simulink model "afe_inv_psm_param"  (R2026b)
settings: Solver=ode23t  StopTime=param.sim.simlength  FixedStep=tc  MaxStep=param.glb_time.tc  RelTol=1e-4
values from neighbouring files (symbols this model uses):
  param = add_template_extras(param, options)    [init_model.m]
undefined symbols (not defined in the file or in its folder): magnitude, omega_m_bez
libraries: fl_lib x330, nesl_utility x174, igbt_simple_2th_lib x12, moving_average_filter x10, moving_average_filter_cc x8, sl_discontinuities x3, single_phase_transformer_lib x3, linear_double_integrator_observer_ccaller x2, discrete_time_low_pass_filter x2, threephase_inductor_lib x2, three_phase_pwm_modulator x2, three_phase_inverter_ideal_switch_based_model x2
(part 8 of 13)

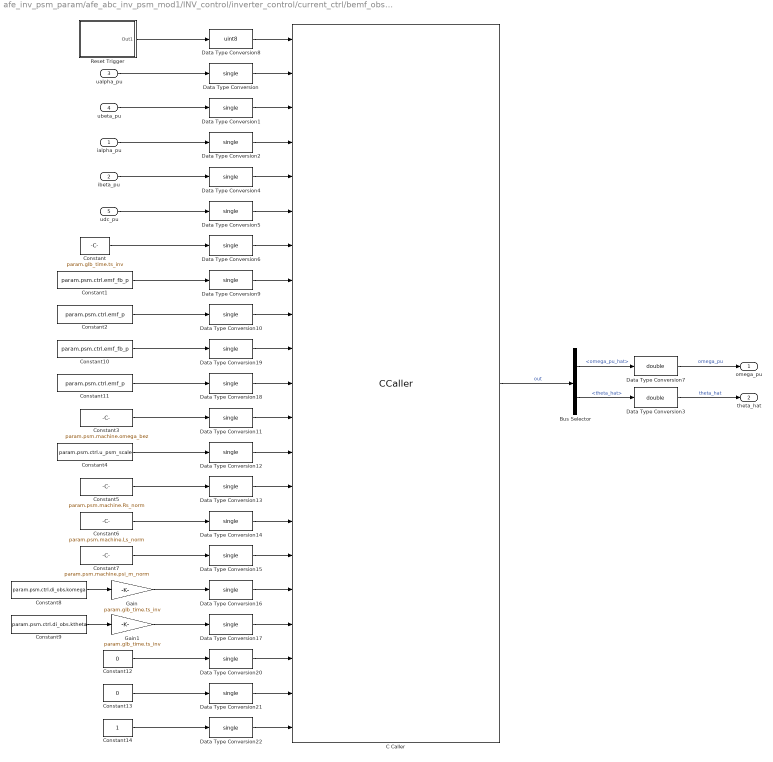
== system afe_inv_psm_param/afe_abc_inv_psm_mod1/INV_control/inverter_control/current_ctrl/bemf_observer/bemf_observer_ccaller ==
  ialpha_pu : Inport
  ibeta_pu : Inport  Port=2
  ualpha_pu : Inport  Port=3
  ubeta_pu : Inport  Port=4
  udc_pu : Inport  Port=5
  Bus Selector : BusSelector  OutputSignals=omega_pu_hat,theta_hat
  C Caller : CCaller  FunctionName=bemf_obsv_process_simulink  PortSpecificationStruct="%)30     .    N\"8   8    (     @         %    \"    !8    !     0         %  0 \"0    $    _    07)G3F%M90  4&]R=$YA;64 4V-O<&4     26YD97@     5'EP90      4VEZ90      27-';&]B86P   X    P    !@    @    $          4    (     0    ,    !         !   P!O=70 #@   #     &    \"     0         !0    @    !     P    $         $  # &]U=  .    .     8    (    !          %    \"     $    &     0         0  ...(+12985 chars)"
  Constant : Constant  Value=param.glb_time.ts_inv
  Constant1 : Constant  Value=param.psm.ctrl.emf_fb_p
  Constant10 : Constant  Value=param.psm.ctrl.emf_fb_p
  Constant11 : Constant  Value=param.psm.ctrl.emf_p
  Constant12 : Constant  Value=0
  Constant13 : Constant  Value=0
  Constant14 : Constant
  Constant2 : Constant  Value=param.psm.ctrl.emf_p
  Constant3 : Constant  Value=param.psm.machine.omega_bez
  Constant4 : Constant  Value=param.psm.ctrl.u_psm_scale
  Constant5 : Constant  Value=param.psm.machine.Rs_norm
  Constant6 : Constant  Value=param.psm.machine.Ls_norm
  Constant7 : Constant  Value=param.psm.machine.psi_m_norm
  Constant8 : Constant  Value=param.psm.ctrl.di_obs.komega
  Constant9 : Constant  Value=param.psm.ctrl.di_obs.ktheta
  Data Type Conversion{,1..2,4..6,9..22} (20 alike) : DataTypeConversion  OutDataTypeStr=single  SaturateOnIntegerOverflow=off  RndMeth=Floor
  Data Type Conversion3 : DataTypeConversion  OutDataTypeStr=double  SaturateOnIntegerOverflow=off  RndMeth=Floor
  Data Type Conversion7 : DataTypeConversion  OutDataTypeStr=double  SaturateOnIntegerOverflow=off  RndMeth=Floor
  Data Type Conversion8 : DataTypeConversion  OutDataTypeStr=uint8  SaturateOnIntegerOverflow=off  RndMeth=Floor
  Gain : Gain  Gain=param.glb_time.ts_inv
  Gain1 : Gain  Gain=param.glb_time.ts_inv
  Reset Trigger : Subsystem
  omega_pu : Outport
  theta_hat : Outport  Port=2
  wires:
  Data Type Conversion5/1 -> C Caller/6
  Data Type Conversion/1 -> C Caller/2
  C Caller/1 -> Bus Selector/1  "out"
  Data Type Conversion1/1 -> C Caller/3
  Data Type Conversion4/1 -> C Caller/5
  Data Type Conversion2/1 -> C Caller/4
  Data Type Conversion6/1 -> C Caller/7
  Bus Selector/2 -> Data Type Conversion3/1  "<theta_hat>"
  Bus Selector/1 -> Data Type Conversion7/1  "<omega_pu_hat>"
  Data Type Conversion7/1 -> omega_pu/1  "omega_pu"
  Data Type Conversion3/1 -> theta_hat/1  "theta_hat"
  Data Type Conversion8/1 -> C Caller/1
  Data Type Conversion9/1 -> C Caller/8
  Data Type Conversion10/1 -> C Caller/9
  Data Type Conversion19/1 -> C Caller/10
  Data Type Conversion18/1 -> C Caller/11
  Data Type Conversion11/1 -> C Caller/12
  Data Type Conversion12/1 -> C Caller/13
  Data Type Conversion13/1 -> C Caller/14
  Data Type Conversion14/1 -> C Caller/15
  Data Type Conversion15/1 -> C Caller/16
  Data Type Conversion16/1 -> C Caller/17
  Data Type Conversion17/1 -> C Caller/18
  Data Type Conversion20/1 -> C Caller/19
  Data Type Conversion21/1 -> C Caller/20
  Data Type Conversion22/1 -> C Caller/21
  Constant14/1 -> Data Type Conversion22/1
  Constant13/1 -> Data Type Conversion21/1
  Constant12/1 -> Data Type Conversion20/1
  Constant9/1 -> Gain1/1
  Constant8/1 -> Gain/1
  Constant7/1 -> Data Type Conversion15/1
  Constant6/1 -> Data Type Conversion14/1
  Constant5/1 -> Data Type Conversion13/1
  Constant4/1 -> Data Type Conversion12/1
  Constant3/1 -> Data Type Conversion11/1
  Constant11/1 -> Data Type Conversion18/1
  Constant10/1 -> Data Type Conversion19/1
  Constant2/1 -> Data Type Conversion10/1
  Constant1/1 -> Data Type Conversion9/1
  Constant/1 -> Data Type Conversion6/1
  ibeta_pu/1 -> Data Type Conversion4/1
  ialpha_pu/1 -> Data Type Conversion2/1
  ubeta_pu/1 -> Data Type Conversion1/1
  ualpha_pu/1 -> Data Type Conversion/1
  Reset Trigger/1(Out1) -> Data Type Conversion8/1
  udc_pu/1 -> Data Type Conversion5/1
  Gain/1 -> Data Type Conversion16/1
  Gain1/1 -> Data Type Conversion17/1

== system afe_inv_psm_param/afe_abc_inv_psm_mod1/INV_control/inverter_control/current_ctrl/current_ctrl/MTPA _mod1 ==
  iq_ref : Inport
  Gain1 : Gain  Gain=1/(param.psm.machine.Ld_norm - param.psm.machine.Lq_norm)/2
  Gain2 : Gain  Gain=1/(param.psm.machine.Ld_norm - param.psm.machine.Lq_norm)/2
  Gain3 : Gain  Gain=-1
  Math Function1 : Math  Operator=magnitude^2  SignedPower=on
  Math Function4 : Math  Operator=magnitude^2  SignedPower=on
  Sqrt : Sqrt
  Sum : Sum  Inputs=|++
  Sum1 : Sum  Inputs=|-+
  id_ref_pu < x < 0 : Saturate  UpperLimit=0  LowerLimit=-param.psm.ctrl.id_lim
  Id_ref_mtpa : Outport  VectorParamsAs1DForOutWhenUnconnected=off
  wires:
  Sum1/1 -> Gain3/1
  id_ref_pu < x < 0/1 -> Id_ref_mtpa/1
  Math Function4/1 -> Sum/1
  Math Function1/1 -> Sum/2
  Gain1/1 -> Math Function4/1
  Sum/1 -> Sqrt/1
  Sqrt/1 -> Sum1/2
  iq_ref/1 -> Math Function1/1
  Gain2/1 -> Sum1/1
  [motor_speed_pu_ctrl_mod1] -> Gain1/1, Gain2/1
  Gain3/1 -> id_ref_pu < x < 0/1

== system afe_inv_psm_param/afe_abc_inv_psm_mod1/INV_control/inverter_control/current_ctrl/current_ctrl/dq_pi_with_vector_antiwindup mod1 ==
  id_ref : Inport
  id : Inport  Port=2
  iq_ref : Inport  Port=3
  iq : Inport  Port=4
  udc_pu : Inport  Port=5
  Variant Source : VariantSource  VariantControls={param.psm.impl.use_current_controller_from_simulink_module_1 == 1, param.psm.impl.use_current_controller_from_ccaller_module_1 == 1}
  Variant Source1 : VariantSource  VariantControls={param.psm.impl.use_current_controller_from_simulink_module_1 == 1, param.psm.impl.use_current_controller_from_ccaller_module_1 == 1}
  dq_vector_pi : Subsystem
  dq_vector_pi_ccaller : Subsystem
  simulink/Ccaller VectorPI : Scope  NumInputPorts=2
      settings: ActiveDisplayYMinimum=-0.12579688616096973  ActiveDisplayYMaximum=0.43534495122730732
  ctrl_d_u : Outport
  ctrl_q_u : Outport  Port=2
  wires:
  id/1 -> dq_vector_pi_ccaller/1(id), dq_vector_pi/1(id)  "id"
  id_ref/1 -> dq_vector_pi_ccaller/2(id_ref), dq_vector_pi/2(id_ref)  "id_ref"
  iq/1 -> dq_vector_pi_ccaller/3(iq), dq_vector_pi/3(iq)  "iq"
  iq_ref/1 -> dq_vector_pi_ccaller/4(iq_ref), dq_vector_pi/4(iq_ref)  "iq_ref"
  dq_vector_pi/1(md_sat) -> Variant Source/1
  dq_vector_pi_ccaller/2(uq_ctrl_out) -> Variant Source1/2
  dq_vector_pi/2(mq_sat) -> Variant Source1/1
  dq_vector_pi_ccaller/1(ud_ctrl_out) -> Variant Source/2
  Variant Source/1 -> ctrl_d_u/1, simulink/Ccaller VectorPI/1  "ctrl_d_u"
  Variant Source1/1 -> simulink/Ccaller VectorPI/2, ctrl_q_u/1  "ctrl_q_u"
  udc_pu/1 -> dq_vector_pi_ccaller/5(udc_pu)

== system afe_inv_psm_param/afe_abc_inv_psm_mod1/INV_control/inverter_control/current_ctrl/current_ctrl/id_ref _mod1 ==
  id_mtpa : Inport
  Constant : Constant  Value=0
  Variant Source : VariantSource  VariantControls={param.psm.mode.use_mtpa == 1, param.psm.mode.use_mtpa == 0}
  id_ref : Outport
  wires:
  Variant Source/1 -> id_ref/1
  id_mtpa/1 -> Variant Source/1
  Constant/1 -> Variant Source/2

== system afe_inv_psm_param/afe_abc_inv_psm_mod1/INV_control/inverter_control/current_ctrl/current_ctrl/output voltage transformation ==
  Unit Delay2 : UnitDelay  SampleTime=-1
  Unit Delay3 : UnitDelay  SampleTime=-1
  dq2alphabeta : MATLAB Function  TreatAsAtomicUnit=on
  tag scope: ualpha_pu_mod1=scoped, ubeta_pu_mod1=scoped
  wires:
  [ud_pu_mod1] -> dq2alphabeta/1(d)
  [uq_pu_mod1] -> dq2alphabeta/2(q)
  Unit Delay2/1 -> [ualpha_pu_mod1]
  dq2alphabeta/2(beta) -> Unit Delay3/1
  Unit Delay3/1 -> [ubeta_pu_mod1]
  dq2alphabeta/1(alpha) -> Unit Delay2/1
  [motor_phase_ctrl_mod1] -> dq2alphabeta/3(gamma)

== system afe_inv_psm_param/afe_abc_inv_psm_mod1/INV_control/inverter_control/phase_compensation_1/alignment_ctrl/pi ==
  u_ref : Inport
  u : Inport  Port=2
  1/Ti : Gain  Gain=kp  SaturateOnIntegerOverflow=on  OutDataTypeStr=Inherit: Same as input  ParamDataTypeStr=Inherit: Same as input
  Saturation : Saturate  UpperLimit=lim_up  LowerLimit=lim_down
  Sum1 : Sum  Inputs=+++  SaturateOnIntegerOverflow=on
  Sum2 : Sum  Inputs=-+  SaturateOnIntegerOverflow=on
  Sum3 : Sum  Inputs=-+  SaturateOnIntegerOverflow=on
  Unit Delay4 : UnitDelay  SampleTime=-1
  kp : Gain  Gain=ki  SaturateOnIntegerOverflow=on  OutDataTypeStr=Inherit: Same as input  ParamDataTypeStr=Inherit: Same as input
  y : Outport
  wires:
  1/Ti/1 -> Sum1/1, Sum3/1
  kp/1 -> Sum1/2
  Sum3/1 -> Unit Delay4/1
  Unit Delay4/1 -> Sum1/3
  u_ref/1 -> Sum2/2
  u/1 -> Sum2/1
  Sum2/1 -> kp/1, 1/Ti/1
  Sum1/1 -> Saturation/1
  Saturation/1 -> Sum3/2, y/1

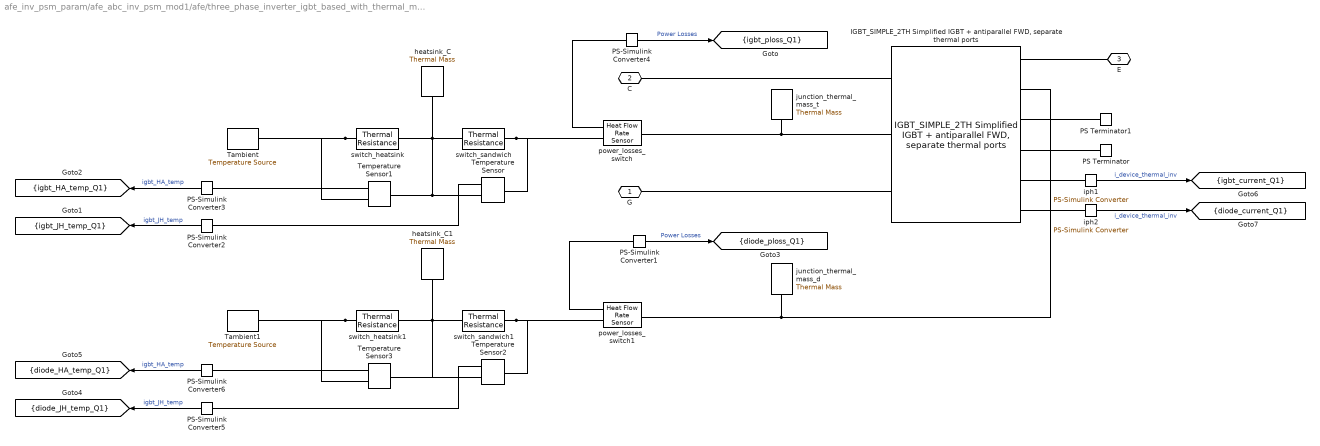
== system afe_inv_psm_param/afe_abc_inv_psm_mod1/afe/three_phase_inverter_igbt_based_with_thermal_model/three_phase_inverter_with_igbt_simple_2th/igbt_simple_1/IGBT_simple ==
  "IGBT_SIMPLE_2TH Simplified IGBT + antiparallel FWD, separate thermal ports" : igbt_simple_2th_lib/IGBT_SIMPLE_2TH Simplified IGBT + antiparallel FWD, separate thermal ports  Vce_sat=vce_sat_m V  Vf=v_gamma_m V  Vth=Vth_gate_m V  Vhyst=Vth_gate_hyst_m V  Eon_ref=Eon_m mJ  Eoff_ref=Eoff_m mJ  Err_ref=Err_m mJ  Ic_ref=Ic_ref_m A  Vdc_ref=Vdc_ref_m V  V_rr_th=Vblock_Errf_m V  Ron=rce_on_m mOhm  Rd=rd_on_m mOhm  Goff=Gce_off_m 1/Ohm  tau_s=time_constant_edge_m us  tau_p=time_constant_ploss_m us  i_specify=off  i_priority=None  i=0 A  i_nominal_specify=off  i_nominal_value=1  i_nominal_unit=A  v_specify=off  v_priority=None  v=0 V  v_nominal_specify=off  v_nominal_value=1  v_nominal_unit=V  i_t_specify=off  i_t_priority=None  i_t=0 A  i_t_nominal_specify=off  i_t_nominal_value=1  i_t_nominal_unit=A  i_d_specify=off  i_d_priority=None  i_d=0 A  i_d_nominal_specify=off  i_d_nominal_value=1  i_d_nominal_unit=A  i_h_specify=off  i_h_priority=None  i_h=0 A  i_h_nominal_specify=off  i_h_nominal_value=1  i_h_nominal_unit=A  i_dh_specify=off  i_dh_priority=None  i_dh=0 A  i_dh_nominal_specify=off  i_dh_nominal_value=1  i_dh_nominal_unit=A  v_h_specify=off  v_h_priority=None  v_h=0 V  v_h_nominal_specify=off  v_h_nominal_value=1  v_h_nominal_unit=V  E_lpt_specify=off  E_lpt_priority=None  E_lpt=0 J  E_lpt_nominal_specify=off  E_lpt_nominal_value=1  E_lpt_nominal_unit=J  E_lpd_specify=off  E_lpd_priority=None  E_lpd=0 J  E_lpd_nominal_specify=off  E_lpd_nominal_value=1  E_lpd_nominal_unit=J  Qt_specify=off  Qt_priority=None  Qt=0 W  Qt_nominal_specify=off  Qt_nominal_value=1  Qt_nominal_unit=W  Qd_specify=off  Qd_priority=None  Qd=0 W  Qd_nominal_specify=off  Qd_nominal_value=1  Qd_nominal_unit=W  E_t_specify=off  E_t_priority=None  E_t=0 J  E_d_specify=off  E_d_priority=None  E_d=0 J
  PS Terminator : fl_lib/Physical Signals/Sinks/PS Terminator
  PS Terminator1 : fl_lib/Physical Signals/Sinks/PS Terminator
  PS-Simulink Converter1 : nesl_utility/PS-Simulink Converter  PhysicalDomain=network_engine_domain  SubClassName=ps_output  LeftPortType=input  RightPortType=output  PseudoPeriodic=off  Frequencies=[]  VectorFormat=1-D array  Unit=J/s  AffineConversion=off
  PS-Simulink Converter{2..3,5..6} (4 alike) : nesl_utility/PS-Simulink Converter  PhysicalDomain=network_engine_domain  SubClassName=ps_output  LeftPortType=input  RightPortType=output  PseudoPeriodic=off  Frequencies=[]  VectorFormat=1-D array  Unit=degC  AffineConversion=off
  PS-Simulink Converter4 : nesl_utility/PS-Simulink Converter  PhysicalDomain=network_engine_domain  SubClassName=ps_output  LeftPortType=input  RightPortType=output  PseudoPeriodic=off  Frequencies=[]  VectorFormat=1-D array  Unit=J/s  AffineConversion=off
  Tambient : fl_lib/Thermal/Thermal Sources/Temperature Source  temperature=Tambient_m degC
  Tambient1 : fl_lib/Thermal/Thermal Sources/Temperature Source  temperature=Tambient_m degC
  Temperature Sensor{,1..3} (4 alike) : fl_lib/Thermal/Thermal Sensors/Temperature Sensor  temperature_measure=foundation.enum.MeasurementReference.difference
  heatsink_C : fl_lib/Thermal/Thermal Elements/Thermal Mass  mass_type=foundation.enum.constant_variable.constant  mass=mass_heatsink_m kg  sp_heat=specific_heat_m J/(K*kg)  mass_min=1e-6 kg  num_ports=foundation.enum.numPorts2.one  m_specify=off  m_priority=High  m=1 kg  m_nominal_specify=off  m_nominal_value=1  m_nominal_unit=kg  T_specify=on  T_priority=High  T=Tambient_m degC  T_nominal_specify=off  T_nominal_value=1  T_nominal_unit=K  Q_specify=off  Q_priority=High  Q=0 W  Q_nominal_specify=off  Q_nominal_value=1  Q_nominal_unit=W
  heatsink_C1 : fl_lib/Thermal/Thermal Elements/Thermal Mass  mass_type=foundation.enum.constant_variable.constant  mass=mass_heatsink_m kg  sp_heat=specific_heat_m J/(K*kg)  mass_min=1e-6 kg  num_ports=foundation.enum.numPorts2.one  m_specify=off  m_priority=High  m=1 kg  m_nominal_specify=off  m_nominal_value=1  m_nominal_unit=kg  T_specify=on  T_priority=High  T=Tambient_m degC  T_nominal_specify=off  T_nominal_value=1  T_nominal_unit=K  Q_specify=off  Q_priority=High  Q=0 W  Q_nominal_specify=off  Q_nominal_value=1  Q_nominal_unit=W
  iph1 : nesl_utility/PS-Simulink Converter  PhysicalDomain=network_engine_domain  SubClassName=ps_output  LeftPortType=input  RightPortType=output  PseudoPeriodic=off  Frequencies=[]  VectorFormat=1-D array  Unit=A  AffineConversion=off
  iph2 : nesl_utility/PS-Simulink Converter  PhysicalDomain=network_engine_domain  SubClassName=ps_output  LeftPortType=input  RightPortType=output  PseudoPeriodic=off  Frequencies=[]  VectorFormat=1-D array  Unit=A  AffineConversion=off
  junction_thermal_mass_d : fl_lib/Thermal/Thermal Elements/Thermal Mass  mass_type=foundation.enum.constant_variable.constant  mass=JunctionTermalMass_m/specific_heat_m kg  sp_heat=specific_heat_m J/(K*kg)  mass_min=1e-6 kg  num_ports=foundation.enum.numPorts2.one  m_specify=off  m_priority=High  m=1 kg  m_nominal_specify=off  m_nominal_value=1  m_nominal_unit=kg  T_specify=on  T_priority=High  T=Tambient_m degC  T_nominal_specify=off  T_nominal_value=1  T_nominal_unit=K  Q_specify=off  Q_priority=High  Q=0 W  Q_nominal_specify=off  Q_nominal_value=1  Q_nominal_unit=W
  junction_thermal_mass_t : fl_lib/Thermal/Thermal Elements/Thermal Mass  mass_type=foundation.enum.constant_variable.constant  mass=JunctionTermalMass_m/specific_heat_m kg  sp_heat=specific_heat_m J/(K*kg)  mass_min=1e-6 kg  num_ports=foundation.enum.numPorts2.one  m_specify=off  m_priority=High  m=1 kg  m_nominal_specify=off  m_nominal_value=1  m_nominal_unit=kg  T_specify=on  T_priority=High  T=Tambient_m degC  T_nominal_specify=off  T_nominal_value=1  T_nominal_unit=K  Q_specify=off  Q_priority=High  Q=0 W  Q_nominal_specify=off  Q_nominal_value=1  Q_nominal_unit=W
  power_losses_switch : fl_lib/Thermal/Thermal Sensors/Heat Flow Rate Sensor
  power_losses_switch1 : fl_lib/Thermal/Thermal Sensors/Heat Flow Rate Sensor
  switch_heatsink : fl_lib/Thermal/Thermal Elements/Thermal Resistance  resistance=rth_switch_HA_m K/W  T_specify=off  T_priority=High  T=0 deltadegC  T_nominal_specify=off  T_nominal_value=1  T_nominal_unit=K  Q_specify=off  Q_priority=None  Q=0 W  Q_nominal_specify=off  Q_nominal_value=1  Q_nominal_unit=W
  switch_heatsink1 : fl_lib/Thermal/Thermal Elements/Thermal Resistance  resistance=rth_diode_HA_m K/W  T_specify=off  T_priority=High  T=0 deltadegC  T_nominal_specify=off  T_nominal_value=1  T_nominal_unit=K  Q_specify=off  Q_priority=None  Q=0 W  Q_nominal_specify=off  Q_nominal_value=1  Q_nominal_unit=W
  switch_sandwich : fl_lib/Thermal/Thermal Elements/Thermal Resistance  resistance=rth_switch_JH_m K/W  T_specify=off  T_priority=High  T=0 degC  T_nominal_specify=off  T_nominal_value=1  T_nominal_unit=K  Q_specify=off  Q_priority=None  Q=0 W  Q_nominal_specify=off  Q_nominal_value=1  Q_nominal_unit=W
  switch_sandwich1 : fl_lib/Thermal/Thermal Elements/Thermal Resistance  resistance=rth_diode_JH_m K/W  T_specify=off  T_priority=High  T=0 degC  T_nominal_specify=off  T_nominal_value=1  T_nominal_unit=K  Q_specify=off  Q_priority=None  Q=0 W  Q_nominal_specify=off  Q_nominal_value=1  Q_nominal_unit=W
  G : PMIOPort  Side=Left
  C : PMIOPort  Port=2  Side=Left
  E : PMIOPort  Port=3  Side=Right
  tag scope: diode_HA_temp_Q1=scoped, diode_JH_temp_Q1=scoped, diode_current_Q1=scoped, diode_ploss_Q1=scoped, igbt_HA_temp_Q1=scoped, igbt_JH_temp_Q1=scoped, igbt_current_Q1=scoped, igbt_ploss_Q1=scoped
  wires:
  PS-Simulink Converter3/1 -> [igbt_HA_temp_Q1]  "igbt_HA_temp"
  PS-Simulink Converter4/1 -> [igbt_ploss_Q1]  "Power Losses"
  PS-Simulink Converter2/1 -> [igbt_JH_temp_Q1]  "igbt_JH_temp"
  PS-Simulink Converter1/1 -> [diode_ploss_Q1]  "Power Losses"
  PS-Simulink Converter5/1 -> [diode_JH_temp_Q1]  "igbt_JH_temp"
  PS-Simulink Converter6/1 -> [diode_HA_temp_Q1]  "igbt_HA_temp"
  iph1/1 -> [igbt_current_Q1]  "i_device_thermal_inv"
  iph2/1 -> [diode_current_Q1]  "i_device_thermal_inv"
  connections:
  Temperature Sensor/RConn2 -- PS-Simulink Converter2/LConn1
  "IGBT_SIMPLE_2TH Simplified IGBT + antiparallel FWD, separate thermal ports"/LConn2 -- junction_thermal_mass_t/LConn1 -- power_losses_switch/LConn1
  Temperature Sensor1/RConn2 -- PS-Simulink Converter3/LConn1
  Temperature Sensor1/LConn1 -- Temperature Sensor/RConn1 -- switch_heatsink/LConn1 -- heatsink_C/LConn1 -- switch_sandwich/RConn1
  switch_heatsink/RConn1 -- Tambient/LConn1 -- Temperature Sensor1/RConn1
  switch_sandwich/LConn1 -- power_losses_switch/RConn2 -- Temperature Sensor/LConn1
  "IGBT_SIMPLE_2TH Simplified IGBT + antiparallel FWD, separate thermal ports"/RConn1 -- E/RConn1
  "IGBT_SIMPLE_2TH Simplified IGBT + antiparallel FWD, separate thermal ports"/LConn1 -- C/RConn1
  "IGBT_SIMPLE_2TH Simplified IGBT + antiparallel FWD, separate thermal ports"/LConn3 -- G/RConn1
  switch_heatsink1/LConn1 -- switch_sandwich1/RConn1 -- heatsink_C1/LConn1 -- Temperature Sensor2/RConn1 -- Temperature Sensor3/LConn1
  switch_heatsink1/RConn1 -- Temperature Sensor3/RConn1 -- Tambient1/LConn1
  switch_sandwich1/LConn1 -- Temperature Sensor2/LConn1 -- power_losses_switch1/RConn2
  Temperature Sensor3/RConn2 -- PS-Simulink Converter6/LConn1
  Temperature Sensor2/RConn2 -- PS-Simulink Converter5/LConn1
  power_losses_switch1/LConn1 -- "IGBT_SIMPLE_2TH Simplified IGBT + antiparallel FWD, separate thermal ports"/RConn2 -- junction_thermal_mass_d/LConn1
  "IGBT_SIMPLE_2TH Simplified IGBT + antiparallel FWD, separate thermal ports"/RConn5 -- iph1/LConn1
  "IGBT_SIMPLE_2TH Simplified IGBT + antiparallel FWD, separate thermal ports"/RConn6 -- iph2/LConn1
  PS Terminator1/LConn1 -- "IGBT_SIMPLE_2TH Simplified IGBT + antiparallel FWD, separate thermal ports"/RConn3
  PS Terminator/LConn1 -- "IGBT_SIMPLE_2TH Simplified IGBT + antiparallel FWD, separate thermal ports"/RConn4
  PS-Simulink Converter4/LConn1 -- power_losses_switch/RConn1
  PS-Simulink Converter1/LConn1 -- power_losses_switch1/RConn1

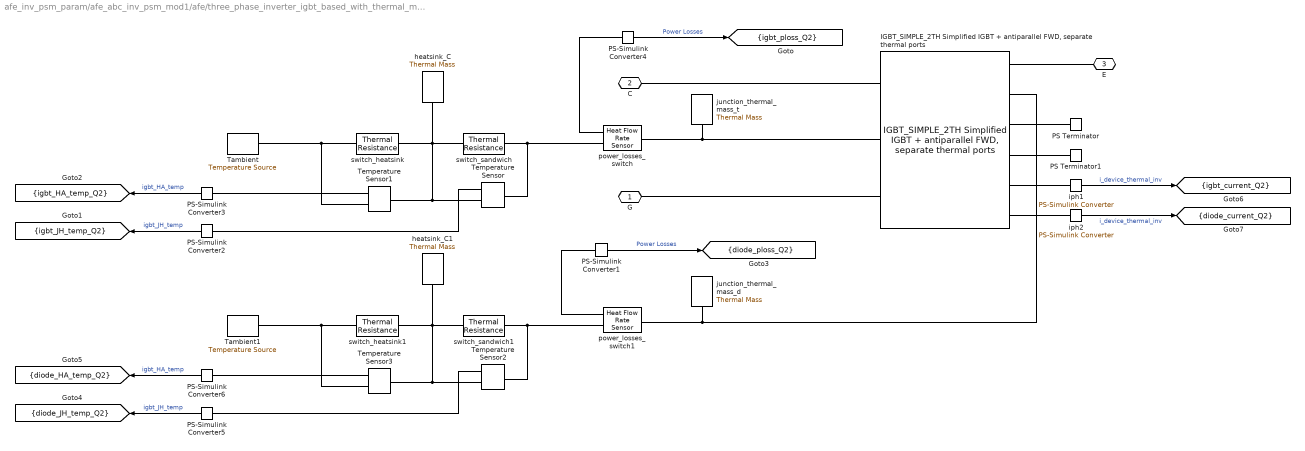
== system afe_inv_psm_param/afe_abc_inv_psm_mod1/afe/three_phase_inverter_igbt_based_with_thermal_model/three_phase_inverter_with_igbt_simple_2th/igbt_simple_2/IGBT_simple ==
  "IGBT_SIMPLE_2TH Simplified IGBT + antiparallel FWD, separate thermal ports" : igbt_simple_2th_lib/IGBT_SIMPLE_2TH Simplified IGBT + antiparallel FWD, separate thermal ports  Vce_sat=vce_sat_m V  Vf=v_gamma_m V  Vth=Vth_gate_m V  Vhyst=Vth_gate_hyst_m V  Eon_ref=Eon_m mJ  Eoff_ref=Eoff_m mJ  Err_ref=Err_m mJ  Ic_ref=Ic_ref_m A  Vdc_ref=Vdc_ref_m V  V_rr_th=Vblock_Errf_m V  Ron=rce_on_m mOhm  Rd=rd_on_m mOhm  Goff=Gce_off_m 1/Ohm  tau_s=time_constant_edge_m us  tau_p=time_constant_ploss_m us  i_specify=off  i_priority=None  i=0 A  i_nominal_specify=off  i_nominal_value=1  i_nominal_unit=A  v_specify=off  v_priority=None  v=0 V  v_nominal_specify=off  v_nominal_value=1  v_nominal_unit=V  i_t_specify=off  i_t_priority=None  i_t=0 A  i_t_nominal_specify=off  i_t_nominal_value=1  i_t_nominal_unit=A  i_d_specify=off  i_d_priority=None  i_d=0 A  i_d_nominal_specify=off  i_d_nominal_value=1  i_d_nominal_unit=A  i_h_specify=off  i_h_priority=None  i_h=0 A  i_h_nominal_specify=off  i_h_nominal_value=1  i_h_nominal_unit=A  i_dh_specify=off  i_dh_priority=None  i_dh=0 A  i_dh_nominal_specify=off  i_dh_nominal_value=1  i_dh_nominal_unit=A  v_h_specify=off  v_h_priority=None  v_h=0 V  v_h_nominal_specify=off  v_h_nominal_value=1  v_h_nominal_unit=V  E_lpt_specify=off  E_lpt_priority=None  E_lpt=0 J  E_lpt_nominal_specify=off  E_lpt_nominal_value=1  E_lpt_nominal_unit=J  E_lpd_specify=off  E_lpd_priority=None  E_lpd=0 J  E_lpd_nominal_specify=off  E_lpd_nominal_value=1  E_lpd_nominal_unit=J  Qt_specify=off  Qt_priority=None  Qt=0 W  Qt_nominal_specify=off  Qt_nominal_value=1  Qt_nominal_unit=W  Qd_specify=off  Qd_priority=None  Qd=0 W  Qd_nominal_specify=off  Qd_nominal_value=1  Qd_nominal_unit=W  E_t_specify=off  E_t_priority=None  E_t=0 J  E_d_specify=off  E_d_priority=None  E_d=0 J
  PS Terminator : fl_lib/Physical Signals/Sinks/PS Terminator
  PS Terminator1 : fl_lib/Physical Signals/Sinks/PS Terminator
  PS-Simulink Converter1 : nesl_utility/PS-Simulink Converter  PhysicalDomain=network_engine_domain  SubClassName=ps_output  LeftPortType=input  RightPortType=output  PseudoPeriodic=off  Frequencies=[]  VectorFormat=1-D array  Unit=J/s  AffineConversion=off
  PS-Simulink Converter{2..3,5..6} (4 alike) : nesl_utility/PS-Simulink Converter  PhysicalDomain=network_engine_domain  SubClassName=ps_output  LeftPortType=input  RightPortType=output  PseudoPeriodic=off  Frequencies=[]  VectorFormat=1-D array  Unit=degC  AffineConversion=off
  PS-Simulink Converter4 : nesl_utility/PS-Simulink Converter  PhysicalDomain=network_engine_domain  SubClassName=ps_output  LeftPortType=input  RightPortType=output  PseudoPeriodic=off  Frequencies=[]  VectorFormat=1-D array  Unit=J/s  AffineConversion=off
  Tambient : fl_lib/Thermal/Thermal Sources/Temperature Source  temperature=Tambient_m degC
  Tambient1 : fl_lib/Thermal/Thermal Sources/Temperature Source  temperature=Tambient_m degC
  Temperature Sensor{,1..3} (4 alike) : fl_lib/Thermal/Thermal Sensors/Temperature Sensor  temperature_measure=foundation.enum.MeasurementReference.difference
  heatsink_C : fl_lib/Thermal/Thermal Elements/Thermal Mass  mass_type=foundation.enum.constant_variable.constant  mass=mass_heatsink_m kg  sp_heat=specific_heat_m J/(K*kg)  mass_min=1e-6 kg  num_ports=foundation.enum.numPorts2.one  m_specify=off  m_priority=High  m=1 kg  m_nominal_specify=off  m_nominal_value=1  m_nominal_unit=kg  T_specify=on  T_priority=High  T=Tambient_m degC  T_nominal_specify=off  T_nominal_value=1  T_nominal_unit=K  Q_specify=off  Q_priority=High  Q=0 W  Q_nominal_specify=off  Q_nominal_value=1  Q_nominal_unit=W
  heatsink_C1 : fl_lib/Thermal/Thermal Elements/Thermal Mass  mass_type=foundation.enum.constant_variable.constant  mass=mass_heatsink_m kg  sp_heat=specific_heat_m J/(K*kg)  mass_min=1e-6 kg  num_ports=foundation.enum.numPorts2.one  m_specify=off  m_priority=High  m=1 kg  m_nominal_specify=off  m_nominal_value=1  m_nominal_unit=kg  T_specify=on  T_priority=High  T=Tambient_m degC  T_nominal_specify=off  T_nominal_value=1  T_nominal_unit=K  Q_specify=off  Q_priority=High  Q=0 W  Q_nominal_specify=off  Q_nominal_value=1  Q_nominal_unit=W
  iph1 : nesl_utility/PS-Simulink Converter  PhysicalDomain=network_engine_domain  SubClassName=ps_output  LeftPortType=input  RightPortType=output  PseudoPeriodic=off  Frequencies=[]  VectorFormat=1-D array  Unit=A  AffineConversion=off
  iph2 : nesl_utility/PS-Simulink Converter  PhysicalDomain=network_engine_domain  SubClassName=ps_output  LeftPortType=input  RightPortType=output  PseudoPeriodic=off  Frequencies=[]  VectorFormat=1-D array  Unit=A  AffineConversion=off
  junction_thermal_mass_d : fl_lib/Thermal/Thermal Elements/Thermal Mass  mass_type=foundation.enum.constant_variable.constant  mass=JunctionTermalMass_m/specific_heat_m kg  sp_heat=specific_heat_m J/(K*kg)  mass_min=1e-6 kg  num_ports=foundation.enum.numPorts2.one  m_specify=off  m_priority=High  m=1 kg  m_nominal_specify=off  m_nominal_value=1  m_nominal_unit=kg  T_specify=on  T_priority=High  T=Tambient_m degC  T_nominal_specify=off  T_nominal_value=1  T_nominal_unit=K  Q_specify=off  Q_priority=High  Q=0 W  Q_nominal_specify=off  Q_nominal_value=1  Q_nominal_unit=W
  junction_thermal_mass_t : fl_lib/Thermal/Thermal Elements/Thermal Mass  mass_type=foundation.enum.constant_variable.constant  mass=JunctionTermalMass_m/specific_heat_m kg  sp_heat=specific_heat_m J/(K*kg)  mass_min=1e-6 kg  num_ports=foundation.enum.numPorts2.one  m_specify=off  m_priority=High  m=1 kg  m_nominal_specify=off  m_nominal_value=1  m_nominal_unit=kg  T_specify=on  T_priority=High  T=Tambient_m degC  T_nominal_specify=off  T_nominal_value=1  T_nominal_unit=K  Q_specify=off  Q_priority=High  Q=0 W  Q_nominal_specify=off  Q_nominal_value=1  Q_nominal_unit=W
  power_losses_switch : fl_lib/Thermal/Thermal Sensors/Heat Flow Rate Sensor
  power_losses_switch1 : fl_lib/Thermal/Thermal Sensors/Heat Flow Rate Sensor
  switch_heatsink : fl_lib/Thermal/Thermal Elements/Thermal Resistance  resistance=rth_switch_HA_m K/W  T_specify=off  T_priority=High  T=0 deltadegC  T_nominal_specify=off  T_nominal_value=1  T_nominal_unit=K  Q_specify=off  Q_priority=None  Q=0 W  Q_nominal_specify=off  Q_nominal_value=1  Q_nominal_unit=W
  switch_heatsink1 : fl_lib/Thermal/Thermal Elements/Thermal Resistance  resistance=rth_diode_HA_m K/W  T_specify=off  T_priority=High  T=0 deltadegC  T_nominal_specify=off  T_nominal_value=1  T_nominal_unit=K  Q_specify=off  Q_priority=None  Q=0 W  Q_nominal_specify=off  Q_nominal_value=1  Q_nominal_unit=W
  switch_sandwich : fl_lib/Thermal/Thermal Elements/Thermal Resistance  resistance=rth_switch_JH_m K/W  T_specify=off  T_priority=High  T=0 degC  T_nominal_specify=off  T_nominal_value=1  T_nominal_unit=K  Q_specify=off  Q_priority=None  Q=0 W  Q_nominal_specify=off  Q_nominal_value=1  Q_nominal_unit=W
  switch_sandwich1 : fl_lib/Thermal/Thermal Elements/Thermal Resistance  resistance=rth_diode_JH_m K/W  T_specify=off  T_priority=High  T=0 degC  T_nominal_specify=off  T_nominal_value=1  T_nominal_unit=K  Q_specify=off  Q_priority=None  Q=0 W  Q_nominal_specify=off  Q_nominal_value=1  Q_nominal_unit=W
  G : PMIOPort  Side=Left
  C : PMIOPort  Port=2  Side=Left
  E : PMIOPort  Port=3  Side=Right
  tag scope: diode_HA_temp_Q2=scoped, diode_JH_temp_Q2=scoped, diode_current_Q2=scoped, diode_ploss_Q2=scoped, igbt_HA_temp_Q2=scoped, igbt_JH_temp_Q2=scoped, igbt_current_Q2=scoped, igbt_ploss_Q2=scoped
  wires:
  iph2/1 -> [diode_current_Q2]  "i_device_thermal_inv"
  iph1/1 -> [igbt_current_Q2]  "i_device_thermal_inv"
  PS-Simulink Converter6/1 -> [diode_HA_temp_Q2]  "igbt_HA_temp"
  PS-Simulink Converter5/1 -> [diode_JH_temp_Q2]  "igbt_JH_temp"
  PS-Simulink Converter1/1 -> [diode_ploss_Q2]  "Power Losses"
  PS-Simulink Converter2/1 -> [igbt_JH_temp_Q2]  "igbt_JH_temp"
  PS-Simulink Converter4/1 -> [igbt_ploss_Q2]  "Power Losses"
  PS-Simulink Converter3/1 -> [igbt_HA_temp_Q2]  "igbt_HA_temp"
  connections:
  iph2/LConn1 -- "IGBT_SIMPLE_2TH Simplified IGBT + antiparallel FWD, separate thermal ports"/RConn6
  iph1/LConn1 -- "IGBT_SIMPLE_2TH Simplified IGBT + antiparallel FWD, separate thermal ports"/RConn5
  power_losses_switch1/LConn1 -- junction_thermal_mass_d/LConn1 -- "IGBT_SIMPLE_2TH Simplified IGBT + antiparallel FWD, separate thermal ports"/RConn2
  Temperature Sensor2/RConn2 -- PS-Simulink Converter5/LConn1
  Temperature Sensor3/RConn2 -- PS-Simulink Converter6/LConn1
  Temperature Sensor2/LConn1 -- switch_sandwich1/LConn1 -- power_losses_switch1/RConn2
  Temperature Sensor3/RConn1 -- switch_heatsink1/RConn1 -- Tambient1/LConn1
  Temperature Sensor3/LConn1 -- Temperature Sensor2/RConn1 -- switch_sandwich1/RConn1 -- switch_heatsink1/LConn1 -- heatsink_C1/LConn1
  "IGBT_SIMPLE_2TH Simplified IGBT + antiparallel FWD, separate thermal ports"/LConn3 -- G/RConn1
  "IGBT_SIMPLE_2TH Simplified IGBT + antiparallel FWD, separate thermal ports"/LConn1 -- C/RConn1
  "IGBT_SIMPLE_2TH Simplified IGBT + antiparallel FWD, separate thermal ports"/RConn1 -- E/RConn1
  Temperature Sensor/LConn1 -- power_losses_switch/RConn2 -- switch_sandwich/LConn1
  Temperature Sensor1/RConn1 -- Tambient/LConn1 -- switch_heatsink/RConn1
  Temperature Sensor/RConn1 -- Temperature Sensor1/LConn1 -- switch_sandwich/RConn1 -- heatsink_C/LConn1 -- switch_heatsink/LConn1
  Temperature Sensor1/RConn2 -- PS-Simulink Converter3/LConn1
  "IGBT_SIMPLE_2TH Simplified IGBT + antiparallel FWD, separate thermal ports"/LConn2 -- junction_thermal_mass_t/LConn1 -- power_losses_switch/LConn1
  Temperature Sensor/RConn2 -- PS-Simulink Converter2/LConn1
  PS Terminator1/LConn1 -- "IGBT_SIMPLE_2TH Simplified IGBT + antiparallel FWD, separate thermal ports"/RConn4
  PS Terminator/LConn1 -- "IGBT_SIMPLE_2TH Simplified IGBT + antiparallel FWD, separate thermal ports"/RConn3
  PS-Simulink Converter4/LConn1 -- power_losses_switch/RConn1
  PS-Simulink Converter1/LConn1 -- power_losses_switch1/RConn1
